simulink model "F1_Simulator"  (R2026a)
settings: Solver=VariableStepAuto  StopTime=260  MaxStep=0.01
values from neighbouring files (symbols this model uses):
  C = [C; C(1,:)]    [f1_corner_map.m]    (also in f1_lateral_tire_table.m = 1.3; f1_sector_map.m = C([true; hypot(diff(C(:,1)), diff(C(:,2))) > 1e-6], :); f1_sensitivity_sweep.m = {; f1_telemetry.m = C([true; hypot(diff(C(:,1)), diff(C(:,2))) > 1e-6], :))
  m = sU >= d0 & sU <= d1    [f1_corner_map.m]    (also in f1_sector_map.m = dC >= edM(k) & dC <= edM(k+1); f1_speed_profile.m = veh.m)
  normalX = -tangentY    [f1_finish_line_params.m]
  normalY = tangentX    [f1_finish_line_params.m]
  s = cumtrapz(tg, v)    [f1_internal_states.m]    (also in f1_track_animation.m = [0; cumsum(hypot(diff(x), diff(y)))]; f1_track_curvature.m = s_all(keepIdx))
  startX = track(1,1)    [f1_finish_line_params.m]
  startY = track(1,2)    [f1_finish_line_params.m]
  tangentX = dirVec(1)    [f1_finish_line_params.m]
  tangentY = dirVec(2)    [f1_finish_line_params.m]
  trackPsi = psi(idx)    [f1_load_raceline.m]    (also in f1_track_curvature.m = atan2(gradient(trackY), gradient(trackX)))
  trackVref = min(trackVref, vf)    [f1_speed_profile.m]
  trackX = x0    [f1_load_raceline.m]    (also in f1_track_curvature.m = x; silverstone_curvature.mat = [-563.032417564 -561.782952087 -560.539483404 -559.300900612)
  trackY = y0    [f1_load_raceline.m]    (also in f1_track_curvature.m = y; silverstone_curvature.mat = [-515.713759288 -514.151171661 -512.584488731 -511.014091481)
undefined symbols (not defined in the file or in its folder): fp_brk_bore, fp_brk_front, fp_brk_maxT, fp_brk_mu_k, fp_brk_pads, fp_brk_Rm, fp_CdA_corner, fp_CdA_straight, fp_eta_tr, fp_gears, fp_h_cg, fp_mu_brake, fp_mu_pk, fp_mu_trac, fp_N_diff, fp_rho, fp_rpm_dn, fp_rpm_lim_end, fp_rpm_lim_ini, fp_rpm_up, fp_track, pwr, veh
libraries: vehdynlibtire x4, autolibsharedcoupling x3, simulink x1, vehdynlibdriver x1, autolibsharedtransfixedgear x1, autolibshareddiff x1, autolibsharedmappedengines x1, autolibshared x1
(part 3 of 5)

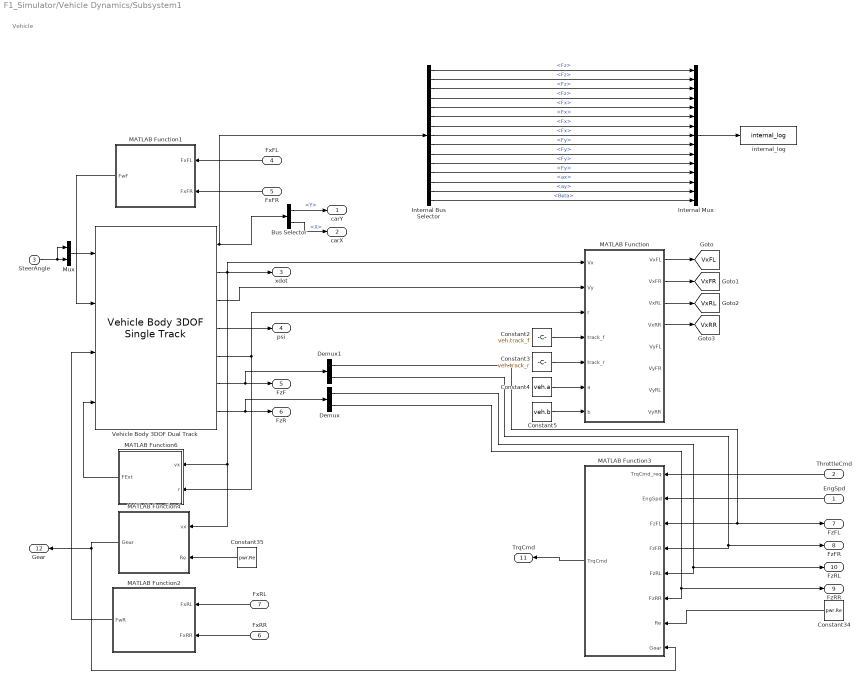
== system F1_Simulator/Vehicle Dynamics/Subsystem1 ==
  note: Vehicle
  EngSpd : Inport
  ThrottleCmd : Inport  Port=2
  SteerAngle : Inport  Port=3
  FxFL : Inport  Port=4
  FxFR : Inport  Port=5
  FxRR : Inport  Port=6
  FxRL : Inport  Port=7
  Bus Selector : BusSelector  OutputSignals=InertFrm.Cg.Disp.Y,InertFrm.Cg.Disp.X
  Constant2 : Constant  Value=veh.track_f
  Constant3 : Constant  Value=veh.track_r
  Constant34 : Constant  Value=pwr.Re
  Constant35 : Constant  Value=pwr.Re
  Constant4 : Constant  Value=veh.a
  Constant5 : Constant  Value=veh.b
  Demux : Demux  Outputs=2
  Demux1 : Demux  Outputs=2
  Internal Bus Selector : BusSelector  OutputSignals=BdyFrm.Forces.Tires.FrntTires.Lft.Fz,BdyFrm.Forces.Tires.FrntTires.Rght.Fz,BdyFrm.Forces.Tires.RearTires.Lft.Fz,BdyFrm.Forces.Tires.RearTires.Rght.Fz,BdyFrm.Forces.Tires.FrntTires.Lft.Fx,BdyFrm.Forces.Tires.FrntTires.Rght.Fx,BdyFrm.Forces.Tires.RearTires.Lft.Fx,BdyFrm.Forces.Tires.RearTires.Rght.Fx,BdyFrm.Forces.Tires.FrntTires.Lft.Fy,BdyFrm.Forces.Tires.FrntTires.Rght.Fy,BdyFrm.Forces.Tires.RearTires.Lft.Fy,BdyFrm.Forces.Tires.RearTires.Rght.Fy,BdyFrm.Cg.Acc.ax,BdyFrm.Cg.Acc.ay,BdyFrm.Cg.Ang.Beta
  Internal Mux : Mux  Inputs=15
  MATLAB Function : MATLAB Function  TreatAsAtomicUnit=on
  MATLAB Function1 : MATLAB Function  TreatAsAtomicUnit=on
  MATLAB Function2 : MATLAB Function  TreatAsAtomicUnit=on
  MATLAB Function3 : MATLAB Function  TreatAsAtomicUnit=on
  MATLAB Function4 : MATLAB Function  TreatAsAtomicUnit=on
  MATLAB Function6 : MATLAB Function  TreatAsAtomicUnit=on
  Mux : Mux  Inputs=2
  Vehicle Body 3DOF Dual Track : autolibshared/Vehicle Body 3DOF Single Track  trackMode=Dual  inputMode=External longitudinal forces  frontSteerMode=on  rearSteerMode=off  extFMode=on  htchFMode=off  extMMode=off  htchMMode=off  windMode=off  extTamb=off  muMode=off  extGndPlnElev=off  extGndPlnRoll=off  extGndPlnPitch=off  extGndPlnDCM=off  extXo=off  extxdoto=off  extYo=off  extydoto=off  extpsio=off  extro=off  aMode=2  NF=2  NR=2  m=veh.m  a=veh.a  b=veh.b  h=veh.cg_height  dh=1  hh=0.2  X_o=startX  xdot_o=0  d=0  hl=0  w=[veh.track_f veh.track_r]  CalphaMode=Mapped slip angle  sigmaMode=on  sigma_f=.1  sigma_r=.1  Cy_f=65e3  Cy_r=80e3  Cy_f_data=Cy_f_tab  alpha_f_brk=alpha_brk  Fz_f_brk="[500\t1.555555555555556e+03\t2.611111111111111e+03\t3.666666666666667e+03\t4.722222222222223e+03\t5.777777777777777e+03\t6.833333333333333e+03\t7.888888888888889e+03\t8.944444444444445e+03\t10000]"  Cy_r_data=Cy_r_tab  alpha_r_brk=alpha_brk  Fz_r_brk="[500\t1.555555555555556e+03\t2.611111111111111e+03\t3.666666666666667e+03\t4.722222222222223e+03\t5.777777777777777e+03\t6.833333333333333e+03\t7.888888888888889e+03\t8.944444444444445e+03\t10000]"  Fznom=tire.Fznom  Y_o=startY  ydot_o=0  Izz=veh.Izz  psi_o=psi_o  r_o=0  Af=aero.Af  Cd=aero.Cd_corner  Cl=aero.Cl  Cpm=0  beta_w=[0 0.01:0.01:0.3]  Cs=[0:0.03:0.9]  Cym=[0 1e-6:0.01:0.3]  Pabs=101325  Tair=288.15  g=9.81  mu=1  GndPlnRoll=0  GndPlnPitch=0  GndPlnElev=0  xdot_tol=.01  Fxtire_sat=7e4  Fytire_sat=7e4  longOff=0  latOff=0  vertOff=veh.cg_height  wrapAng=off
      settings: LibrarySourceBlock=vehdynlibeom/Vehicle Body 3DOF Dual Track
  internal_log : ToWorkspace  VariableName=internal_log  SaveFormat=Timeseries  SampleTime=-1
  carY : Outport
  carX : Outport  Port=2
  xdot : Outport  Port=3
  psi : Outport  Port=4
  FzF : Outport  Port=5
  FzR : Outport  Port=6
  FzFL : Outport  Port=7
  FzFR : Outport  Port=8
  FzRR : Outport  Port=9
  FzRL : Outport  Port=10
  TrqCmd : Outport  Port=11
  Gear : Outport  Port=12
  tag scope: VxFL=global, VxFR=global, VxRL=global, VxRR=global
  wires:
  MATLAB Function/4(VxRR) -> [VxRR]
  MATLAB Function4/1(Gear) -> MATLAB Function3/8(Gear), Gear/1
  EngSpd/1 -> MATLAB Function3/2(EngSpd)
  ThrottleCmd/1 -> MATLAB Function3/1(TrqCmd_req)
  Demux1/2 -> MATLAB Function3/4(FzFR), FzFR/1
  Bus Selector/1 -> carY/1  "<Y>"
  Constant2/1 -> MATLAB Function/4(track_f)
  Vehicle Body 3DOF Dual Track/7 -> FzR/1, Demux/1
  Vehicle Body 3DOF Dual Track/5 -> MATLAB Function6/2(r), MATLAB Function/3(r)
  Vehicle Body 3DOF Dual Track/1 -> Bus Selector/1, Internal Bus Selector/1
  Vehicle Body 3DOF Dual Track/4 -> psi/1
  MATLAB Function/1(VxFL) -> [VxFL]
  Vehicle Body 3DOF Dual Track/2 -> xdot/1, MATLAB Function4/1(vx), MATLAB Function6/1(vx), MATLAB Function/1(Vx)
  Vehicle Body 3DOF Dual Track/6 -> FzF/1, Demux1/1
  FxRL/1 -> MATLAB Function2/1(FxRL)
  Vehicle Body 3DOF Dual Track/3 -> MATLAB Function/2(Vy)
  Demux/2 -> FzRR/1, MATLAB Function3/6(FzRR)
  Constant5/1 -> MATLAB Function/7(b)
  SteerAngle/1 -> Mux/1, Mux/2
  Bus Selector/2 -> carX/1  "<X>"
  MATLAB Function6/1(FExt) -> Vehicle Body 3DOF Dual Track/4
  MATLAB Function2/1(FwR) -> Vehicle Body 3DOF Dual Track/3
  FxFL/1 -> MATLAB Function1/1(FxFL)
  MATLAB Function1/1(FwF) -> Vehicle Body 3DOF Dual Track/2
  Mux/1 -> Vehicle Body 3DOF Dual Track/1
  Constant4/1 -> MATLAB Function/6(a)
  Demux/1 -> FzRL/1, MATLAB Function3/5(FzRL)
  Demux1/1 -> FzFL/1, MATLAB Function3/3(FzFL)
  FxFR/1 -> MATLAB Function1/2(FxFR)
  Constant3/1 -> MATLAB Function/5(track_r)
  MATLAB Function/2(VxFR) -> [VxFR]
  Constant35/1 -> MATLAB Function4/2(Re)
  Constant34/1 -> MATLAB Function3/7(Re)
  MATLAB Function/3(VxRL) -> [VxRL]
  FxRR/1 -> MATLAB Function2/2(FxRR)
  MATLAB Function3/1(TrqCmd) -> TrqCmd/1
  Internal Bus Selector/1 -> Internal Mux/1  "<Fz>"
  Internal Bus Selector/2 -> Internal Mux/2  "<Fz>"
  Internal Bus Selector/3 -> Internal Mux/3  "<Fz>"
  Internal Bus Selector/4 -> Internal Mux/4  "<Fz>"
  Internal Bus Selector/5 -> Internal Mux/5  "<Fx>"
  Internal Bus Selector/6 -> Internal Mux/6  "<Fx>"
  Internal Bus Selector/7 -> Internal Mux/7  "<Fx>"
  Internal Bus Selector/8 -> Internal Mux/8  "<Fx>"
  Internal Bus Selector/9 -> Internal Mux/9  "<Fy>"
  Internal Bus Selector/10 -> Internal Mux/10  "<Fy>"
  Internal Bus Selector/11 -> Internal Mux/11  "<Fy>"
  Internal Bus Selector/12 -> Internal Mux/12  "<Fy>"
  Internal Bus Selector/13 -> Internal Mux/13  "<ax>"
  Internal Bus Selector/14 -> Internal Mux/14  "<ay>"
  Internal Bus Selector/15 -> Internal Mux/15  "<Beta>"
  Internal Mux/1 -> internal_log/1
